simulink model "LMPC_2nd_order_Kang_2"  (R2024b)
settings: Solver=FixedStepAuto  StartTime=0.0  StopTime=10.0  FixedStep=T_sample  RelTol=1e-3
values from neighbouring files (symbols this model uses):
  a = p.x_model(1)    [Run_MPC_For_2nd_order_Plant.m]    (also in Run_MPC_For_2nd_order_Plant_auto_tuning.m = x_model(1))
  b = p.x_model(3)    [Run_MPC_For_2nd_order_Plant.m]    (also in Run_MPC_For_2nd_order_Plant_auto_tuning.m = x_model(3))
  c = p.x_model(2)    [Run_MPC_For_2nd_order_Plant.m]    (also in Run_MPC_For_2nd_order_Plant_auto_tuning.m = x_model(2))
  f0 = p.x_model(4)    [Run_MPC_For_2nd_order_Plant.m]    (also in Run_MPC_For_2nd_order_Plant_auto_tuning.m = x_model(4))
  Q1 = 1    [Run_MPC_For_2nd_order_Plant.m]    (also in Run_MPC_For_2nd_order_Plant_auto_tuning.m)
  Q2 = 0.015    [Run_MPC_For_2nd_order_Plant.m]    (also in Run_MPC_For_2nd_order_Plant_auto_tuning.m = x(1))
  R = 0.1    [Run_MPC_For_2nd_order_Plant.m]    (also in Run_MPC_For_2nd_order_Plant_auto_tuning.m = x(2))
  T_sample = .01    (= 0.01)    [Run_MPC_For_2nd_order_Plant.m]    (also in Run_MPC_For_2nd_order_Plant_auto_tuning.m)
settings Model: Creator=Arrow  LastModifiedBy=sk3547969879
settings OptimizationCC: ReuseModelBlockBuffer=off
settings RTWCC: GPUComputeCapability=3.5

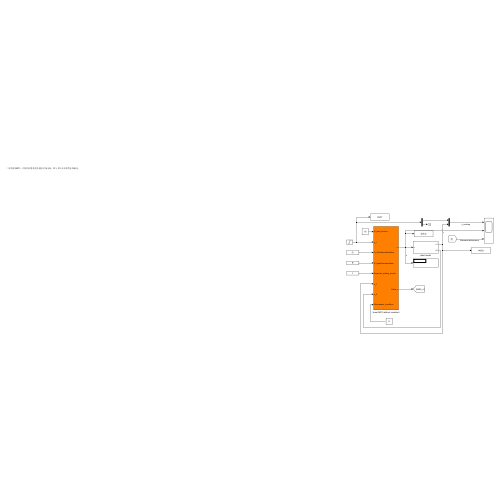
[thumbnail: Simulink's stored preview of the top-level diagram]
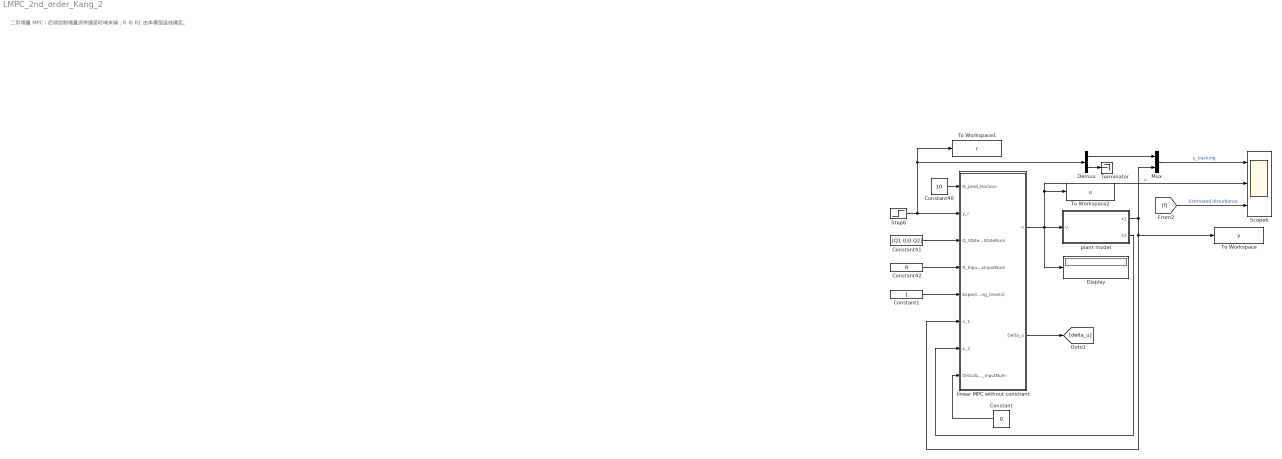
== system LMPC_2nd_order_Kang_2 ==
  note: 二阶增量 MPC：后续控制增量须传播至时域末端；R 与 R1 由本模型连线确定。
  Constant : Constant  Value=0
  Constant1 : Constant
  Constant40 : Constant  Value=10
  Constant41 : Constant  Value=[Q1 0;0 Q2]
  Constant42 : Constant  Value=R
  Demux : Demux  Outputs=2
  Display : Display
  Mux : Mux  Inputs=2
  Scope6 : Scope  NumInputPorts=3
  Step6 : Step  Time=5  Before=[0; 0]  After=[1; 0]  SampleTime=0
  Terminator : Terminator
  To Workspace : ToWorkspace  VariableName=y  SaveFormat=Timeseries  SampleTime=-1
  To Workspace1 : ToWorkspace  VariableName=r  SaveFormat=Timeseries  SampleTime=-1
  To Workspace2 : ToWorkspace  VariableName=u  SaveFormat=Timeseries  SampleTime=-1
  linear MPC without constrant : Subsystem
  plant model : Subsystem
  wires:
  Constant41/1 -> linear MPC without constrant/3(Q_StateNumxStateNum)
  linear MPC without constrant/1(u) -> To Workspace2/1, Scope6/2, Display/1, plant model/1(u)  "u"
  Step6/1 -> To Workspace1/1, Demux/1, linear MPC without constrant/2(y_r)
  Constant42/1 -> linear MPC without constrant/4(R_InputNumxInputNum)
  Mux/1 -> Scope6/1  "y_tracking"
  Constant40/1 -> linear MPC without constrant/1(N_pred_Horizon)
  plant model/2(x2) -> linear MPC without constrant/7(x_2)
  Constant1/1 -> linear MPC without constrant/5(Expected_settling_time(s))
  Demux/1 -> Mux/1
  Demux/2 -> Terminator/1
  plant model/1(x1) -> To Workspace/1, linear MPC without constrant/6(x_1), Mux/2
  linear MPC without constrant/2(Delta_u) -> [delta_u]
  Constant/1 -> linear MPC without constrant/8(Disturbance_InputNum)
  [f] -> Scope6/3  "Estimated disturbance"

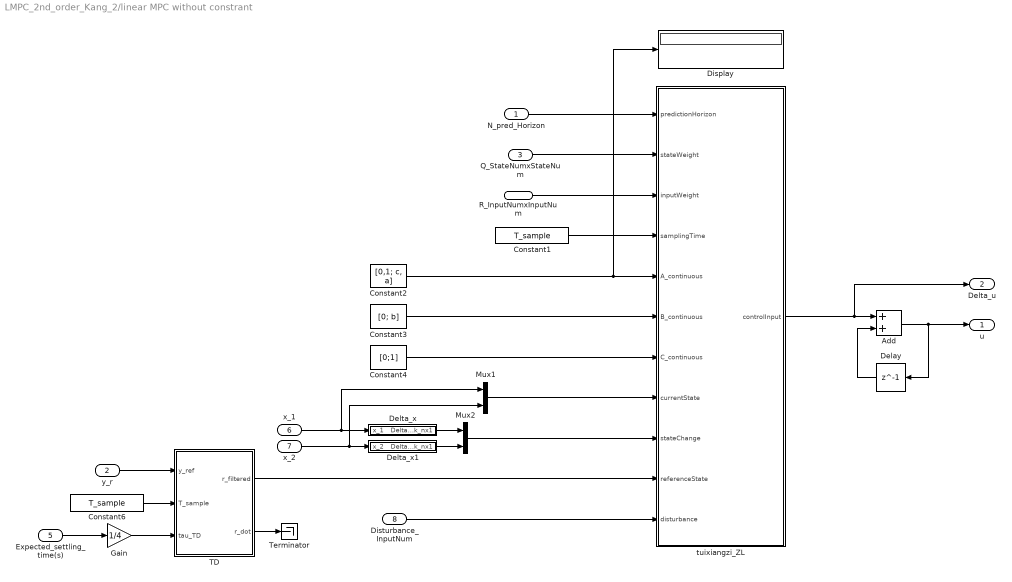
== system LMPC_2nd_order_Kang_2/linear MPC without constrant ==
  N_pred_Horizon : Inport
  y_r : Inport  Port=2
  Q_StateNumxStateNum : Inport  Port=3
  R_InputNumxInputNum : Inport  Port=4
  Expected_settling_time(s) : Inport  Port=5
  x_1 : Inport  Port=6
  x_2 : Inport  Port=7
  Disturbance_InputNum : Inport  Port=8
  Add : Sum
  Constant1 : Constant  Value=T_sample
  Constant2 : Constant  Value=[0,1; c, a]
  Constant3 : Constant  Value=[0; b]
  Constant4 : Constant  Value=[0;1]
  Constant6 : Constant  Value=T_sample
  Delay : Delay  DelayLength=1
  Delta_x : Subsystem
  Delta_x1 : Subsystem
  Display : Display
  Gain : Gain  Gain=1/4
  Mux1 : Mux  Inputs=2
  Mux2 : Mux  Inputs=2
  TD : Subsystem
  Terminator : Terminator
  tuixiangzi_ZL : MATLAB Function  TreatAsAtomicUnit=on
  u : Outport
  Delta_u : Outport  Port=2
  wires:
  tuixiangzi_ZL/1(controlInput) -> Delta_u/1, Add/1
  Constant1/1 -> tuixiangzi_ZL/4(samplingTime)
  Add/1 -> Delay/1, u/1
  Delay/1 -> Add/2
  R_InputNumxInputNum/1 -> tuixiangzi_ZL/3(inputWeight)
  Mux1/1 -> tuixiangzi_ZL/8(currentState)
  x_1/1 -> Delta_x/1(x_1), Mux1/1
  x_2/1 -> Delta_x1/1(x_2), Mux1/2
  Delta_x/1(Delta_Xk_nx1) -> Mux2/1
  Delta_x1/1(Delta_Xk_nx1) -> Mux2/2
  Mux2/1 -> tuixiangzi_ZL/9(stateChange)
  Disturbance_InputNum/1 -> tuixiangzi_ZL/11(disturbance)
  Q_StateNumxStateNum/1 -> tuixiangzi_ZL/2(stateWeight)
  N_pred_Horizon/1 -> tuixiangzi_ZL/1(predictionHorizon)
  Constant2/1 -> Display/1, tuixiangzi_ZL/5(A_continuous)
  Constant3/1 -> tuixiangzi_ZL/6(B_continuous)
  Constant4/1 -> tuixiangzi_ZL/7(C_continuous)
  Constant6/1 -> TD/2(T_sample)
  TD/2(r_dot) -> Terminator/1
  Gain/1 -> TD/3(tau_TD)
  Expected_settling_time(s)/1 -> Gain/1
  y_r/1 -> TD/1(y_ref)
  TD/1(r_filtered) -> tuixiangzi_ZL/10(referenceState)

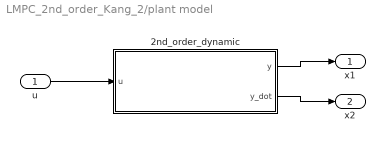
== system LMPC_2nd_order_Kang_2/plant model ==
  u : Inport
  2nd_order_dynamic : Subsystem
  x1 : Outport
  x2 : Outport  Port=2
  wires:
  2nd_order_dynamic/2(y_dot) -> x2/1
  u/1 -> 2nd_order_dynamic/1(u)
  2nd_order_dynamic/1(y) -> x1/1

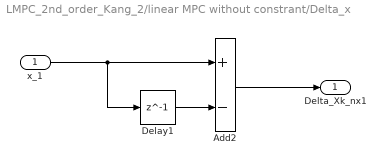
== system LMPC_2nd_order_Kang_2/linear MPC without constrant/Delta_x ==
  x_1 : Inport
  Add2 : Sum  Inputs=+-
  Delay1 : Delay  DelayLength=1  InitialCondition=0
  Delta_Xk_nx1 : Outport
  wires:
  Delay1/1 -> Add2/2
  x_1/1 -> Delay1/1, Add2/1
  Add2/1 -> Delta_Xk_nx1/1

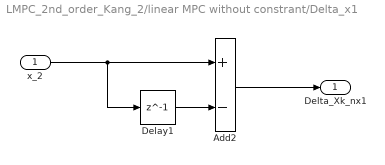
== system LMPC_2nd_order_Kang_2/linear MPC without constrant/Delta_x1 ==
  x_2 : Inport
  Add2 : Sum  Inputs=+-
  Delay1 : Delay  DelayLength=1  InitialCondition=0
  Delta_Xk_nx1 : Outport
  wires:
  Add2/1 -> Delta_Xk_nx1/1
  x_2/1 -> Add2/1, Delay1/1
  Delay1/1 -> Add2/2

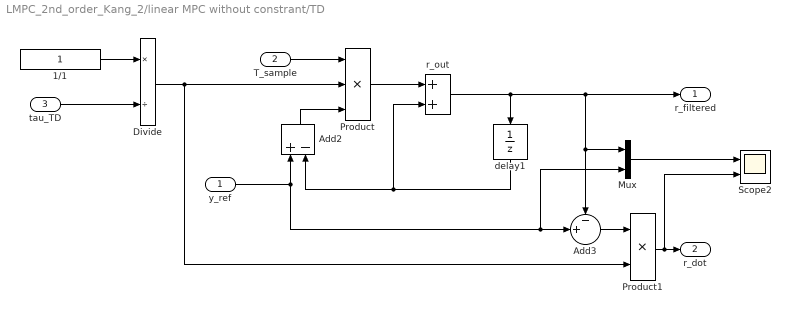
== system LMPC_2nd_order_Kang_2/linear MPC without constrant/TD ==
  y_ref : Inport
  T_sample : Inport  Port=2
  tau_TD : Inport  Port=3
  1/1 : Constant
  Add2 : Sum  Inputs=+-
  Add3 : Sum  Inputs=-+|
  Divide : Product  Inputs=*/
  Mux : Mux  Inputs=2
  Product : Product  Inputs=3  RndMeth=Zero
  Product1 : Product  RndMeth=Zero
  Scope2 : Scope  NumInputPorts=2
  delay1 : UnitDelay  SampleTime=-1  HasFrameUpgradeWarning=on
  r_out : Sum
  r_filtered : Outport  VectorParamsAs1DForOutWhenUnconnected=off
  r_dot : Outport  Port=2  VectorParamsAs1DForOutWhenUnconnected=off
  wires:
  T_sample/1 -> Product/1
  Divide/1 -> Product1/2, Product/2
  Add3/1 -> Product1/1
  r_out/1 -> r_filtered/1, Mux/1, Add3/1, delay1/1
  Add2/1 -> Product/3
  Product1/1 -> Scope2/2, r_dot/1
  delay1/1 -> r_out/2, Add2/2
  y_ref/1 -> Mux/2, Add3/2, Add2/1
  Product/1 -> r_out/1
  Mux/1 -> Scope2/1
  1/1/1 -> Divide/1
  tau_TD/1 -> Divide/2

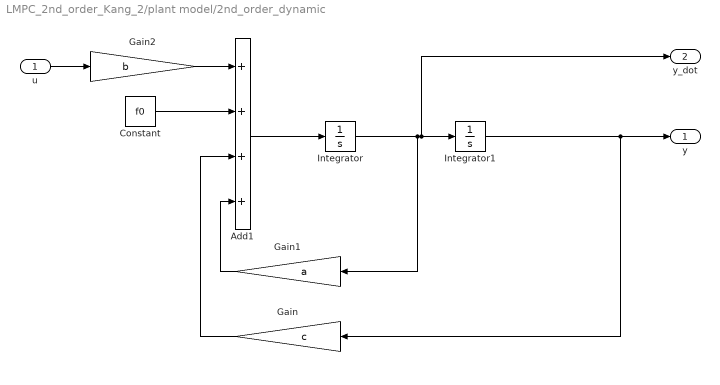
== system LMPC_2nd_order_Kang_2/plant model/2nd_order_dynamic ==
  u : Inport
  Add1 : Sum  Inputs=++++
  Constant : Constant  Value=f0
  Gain : Gain  Gain=c
  Gain1 : Gain  Gain=a
  Gain2 : Gain  Gain=b
  Integrator : Integrator
  Integrator1 : Integrator
  y : Outport
  y_dot : Outport  Port=2
  wires:
  Add1/1 -> Integrator/1
  Gain/1 -> Add1/3
  u/1 -> Gain2/1
  Integrator/1 -> Gain1/1, y_dot/1, Integrator1/1
  Integrator1/1 -> Gain/1, y/1
  Gain2/1 -> Add1/1
  Gain1/1 -> Add1/4
  Constant/1 -> Add1/2

== matlab function LMPC_2nd_order_Kang_2/linear MPC without constrant/tuixiangzi_ZL ==
  data: predictionHorizon input; controlInput output size=1; stateWeight input; inputWeight input; samplingTime input; A_continuous input; B_continuous input; C_continuous input; currentState input; stateChange input; referenceState input; disturbance input
function controlInput = MPC_QP(predictionHorizon, stateWeight, inputWeight, samplingTime, A_continuous, B_continuous, C_continuous, currentState, stateChange, referenceState, disturbance)
% Model Predictive Control (MPC) based on Quadratic Programming (QP)
% 
% Inputs:
% - predictionHorizon: The prediction horizon for MPC.
% - stateWeight: Weight matrix for state deviation in the cost function.
% - inputWeight: Weight matrix for control input in the cost function.
% - samplingTime: Time step for discretization.
% - A_continuous, B_continuous, C_continuous: Continuous-time system matrices.
% - currentState: The current state of the system.
% - stateChange: The difference between the current state and the previous state.
% - referenceState: The desired reference state for the system.
% - disturbance: Estimated disturbance for the system.
%
% Outputs:
% - controlInput: The computed control input based on MPC.

%%%%%%%%%%%%%%%%%%%%%%%%

% Compute the dimension of the state vector
stateDim = size(A_continuous, 1); 

% Discretize the continuous-time system matrices using Euler method
A_discrete = A_continuous .* samplingTime + eye(stateDim);
B_discrete = B_continuous .* samplingTime;
C_discrete = C_continuous .* samplingTime;

% Compute the dimension of the input vector
inputDim = size(B_discrete, 2);

% Construct the extended weight matrices for the entire prediction horizon using the Kronecker product
Q_bar = kron(eye(predictionHorizon), stateWeight);
R_bar = kron(eye(predictionHorizon), inputWeight);

% Pre-compute certain operations to avoid repeated calculations and enhance efficiency
Q_bar_transpose_times_Q_bar = Q_bar' * Q_bar;
R_bar_transpose_times_R_bar = R_bar' * R_bar;

% Use repmat to create a vector by repeating the reference state for the entire prediction horizon
referenceStateAugmented = repmat(referenceState, predictionHorizon, 1);

% Initialization of matrices that will represent the prediction model over the horizon
stateMatrix = [A_discrete; zeros((predictionHorizon-1)*stateDim, stateDim)];
identityMatrix = [eye(stateDim); zeros((predictionHorizon-1)*stateDim, stateDim)];
controlMatrix = [C_discrete; zeros((predictionHorizon-1)*stateDim, inputDim)];
inputMatrix = zeros(predictionHorizon*stateDim, predictionHorizon*inputDim);

% Temporary matrices to assist in constructing the prediction model
tmpMatrix1 = A_discrete;
tmpMatrix2 = C_discrete;

% Build the prediction model matrices over the horizon
for i = 1:predictionHorizon-1
    rows = i*stateDim + (1:stateDim);
    tmpMatrix1 = A_discrete + tmpMatrix1 * A_discrete;
    stateMatrix(rows, :) = tmpMatrix1;
    identityMatrix(rows, :) = eye(stateDim);
    tmpMatrix2 = C_discrete + A_discrete * tmpMatrix2;
    controlMatrix(rows, :) = tmpMatrix2;
end

% Populate the input matrix over the horizon
inputMatrix(1:stateDim, 1:inputDim) = B_discrete;
tmpMatrix3 = B_discrete;

for i = 1:predictionHorizon-1
    rows = i*stateDim + (1:stateDim);
    tmpMatrix3 = B_discrete + A_discrete * tmpMatrix3;
    inputMatrix(rows, 1:inputDim) = tmpMatrix3;
end

% Adjust the input matrix based on the prediction horizon
for j = 1:predictionHorizon-1
    columns = j*inputDim + (1:inputDim);
    start = j*stateDim + 1;
    % 第 j 个增量对所有剩余预测步均有影响。
    stop = predictionHorizon * stateDim;
    inputMatrix(start:stop, columns) = inputMatrix(1:stop-start+1, 1:inputDim);
end

if size(controlMatrix, 2) ~= size(disturbance, 1)
    error('Dimensions of controlMatrix and disturbance do not match for multiplication');
end


% Compute the prediction error over the horizon
errorPrediction = referenceStateAugmented - stateMatrix * stateChange - identityMatrix * currentState - controlMatrix * disturbance;

% Compute the optimal control matrix using the pre-computed matrices
controlMatrixOptimal = inputMatrix' * Q_bar * inputMatrix + R_bar;

% Solve the quadratic program to determine the change in control input over the horizon
deltaControl = controlMatrixOptimal \ inputMatrix' * Q_bar * errorPrediction;

% Return the first control input from the delta control sequence
controlInput = deltaControl(1:inputDim);

end
